simulink model "accelerr_test_drvr"  (Simulink 4.00)
settings: Solver=ode45  StartTime=0.0  StopTime=10.0  RelTol=1e-3
undefined symbols (not defined in the file or in its folder): DCM_B2L, DCM_L2E, skew
settings Model: Creator=mcar  LastModifiedBy=mcar  BlockReductionOpt=off

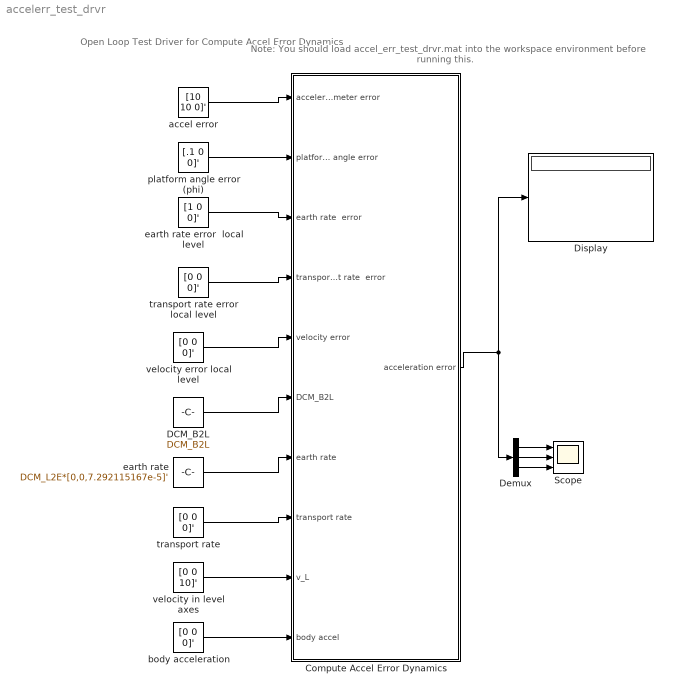
== system accelerr_test_drvr ==
  note: Open Loop Test Driver
      | for Compute Accel Error
      | Dynamics
  note: Note: You should load accel_err_test_drvr.mat into
      | the workspace environment before running this.
  Compute Accel Error Dynamics : Subsystem
      settings: RTWFcnNameOpts=Auto  RTWFileNameOpts=Auto
  DCM_B2L : Constant  Value=DCM_B2L  VectorParams1D=off
  Demux : Demux  Outputs=3  BusSelectionMode=off
  Display : Display
      settings: Format=short
  Scope : Scope  NumInputPorts=3
      settings: TimeRange=auto  YMin=-5~-5~-5  YMax=5~5~5  SaveToWorkspace=off  SaveName=ScopeData  LimitDataPoints=on  MaxDataPoints=5000
  accel error : Constant  Value=[10 10 0]'  VectorParams1D=off
  body acceleration : Constant  Value=[0 0 0]'  VectorParams1D=off
  earth rate : Constant  Value=DCM_L2E*[0,0,7.292115167e-5]'  VectorParams1D=off
  earth rate error  local level : Constant  Value=[1 0 0]'  VectorParams1D=off
  platform angle error (phi) : Constant  Value=[.1 0 0]'  VectorParams1D=off
  transport rate : Constant  Value=[0 0 0]'  VectorParams1D=off
  transport rate error local level : Constant  Value=[0 0 0]'  VectorParams1D=off
  velocity error local level : Constant  Value=[0 0 0]'  VectorParams1D=off
  velocity in level axes : Constant  Value=[0 0 10]'  VectorParams1D=off
  wires:
  body acceleration/1 -> Compute Accel Error Dynamics/10(body accel)
  velocity in level axes/1 -> Compute Accel Error Dynamics/9(v_L)
  transport rate/1 -> Compute Accel Error Dynamics/8(transport rate)
  earth rate/1 -> Compute Accel Error Dynamics/7(earth rate)
  DCM_B2L/1 -> Compute Accel Error Dynamics/6(DCM_B2L)
  velocity error local level/1 -> Compute Accel Error Dynamics/5(velocity error)
  transport rate error local level/1 -> Compute Accel Error Dynamics/4(transport rate  error)
  earth rate error  local level/1 -> Compute Accel Error Dynamics/3(earth rate  error)
  platform angle error (phi)/1 -> Compute Accel Error Dynamics/2(platform  angle error)
  accel error/1 -> Compute Accel Error Dynamics/1(accelerometer error)
  Compute Accel Error Dynamics/1(acceleration error) -> Demux/1, Display/1
  Demux/1 -> Scope/1
  Demux/2 -> Scope/2
  Demux/3 -> Scope/3

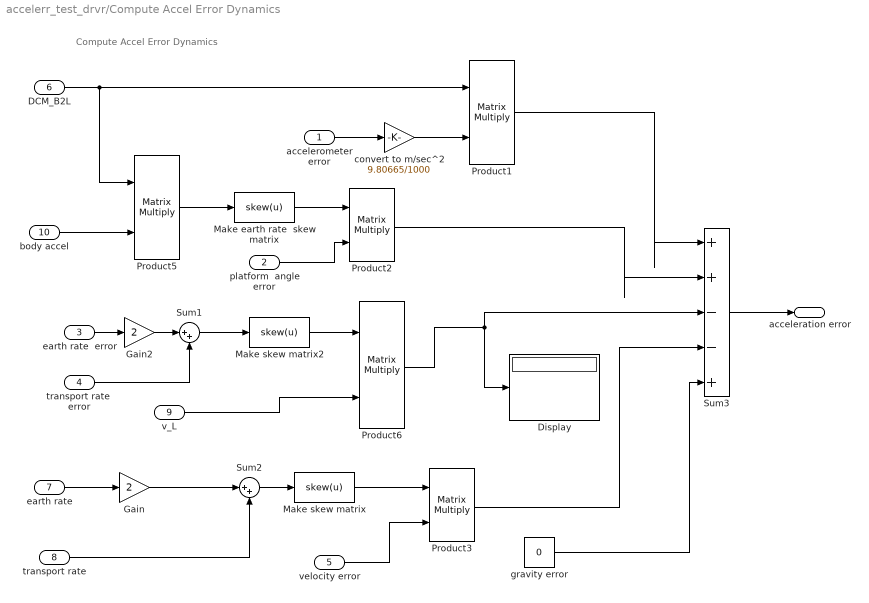
== system accelerr_test_drvr/Compute Accel Error Dynamics ==
  note: Compute Accel Error Dynamics
  accelerometer error : Inport  Port=1
  platform  angle error : Inport  Port=2
  earth rate  error : Inport  Port=3
  transport rate  error : Inport  Port=4
  velocity error : Inport  Port=5
  DCM_B2L : Inport  Port=6
  earth rate : Inport  Port=7
  transport rate : Inport  Port=8
  v_L : Inport  Port=9
  body accel : Inport  Port=10
  Display : Display
      settings: Format=short
  Gain : Gain  Gain=2  Multiplication=Element-wise(K.*u)  SaturateOnIntegerOverflow=on
  Gain2 : Gain  Gain=2  Multiplication=Element-wise(K.*u)  SaturateOnIntegerOverflow=on
  Make earth rate  skew matrix : MATLABFcn  MATLABFcn=skew(u)  OutputDimensions=-1  OutputSignalType=auto  Output1D=off
  Make skew matrix : MATLABFcn  MATLABFcn=skew(u)  OutputDimensions=-1  OutputSignalType=auto  Output1D=off
  Make skew matrix2 : MATLABFcn  MATLABFcn=skew(u)  OutputDimensions=-1  OutputSignalType=auto  Output1D=off
  Product{1..3,5..6} (5 alike) : Product  Inputs=2  Multiplication=Matrix(*)  SaturateOnIntegerOverflow=on
  Sum1 : Sum  Inputs=|++  SaturateOnIntegerOverflow=on
  Sum2 : Sum  Inputs=|++  SaturateOnIntegerOverflow=on
  Sum3 : Sum  Inputs=|++--+  SaturateOnIntegerOverflow=on
  convert to m/sec^2 : Gain  Gain=9.80665/1000  Multiplication=Element-wise(K.*u)  SaturateOnIntegerOverflow=on
  gravity error : Constant  Value=0
  acceleration error : Outport  Port=1
  wires:
  accelerometer error/1 -> convert to m/sec^2/1
  Make earth rate  skew matrix/1 -> Product2/1
  platform  angle error/1 -> Product2/2
  Gain/1 -> Sum2/1
  Sum2/1 -> Make skew matrix/1
  Make skew matrix/1 -> Product3/1
  velocity error/1 -> Product3/2
  earth rate  error/1 -> Gain2/1
  Gain2/1 -> Sum1/1
  transport rate  error/1 -> Sum1/2
  Sum1/1 -> Make skew matrix2/1
  Sum3/1 -> acceleration error/1
  Product1/1 -> Sum3/1
  Product2/1 -> Sum3/2
  gravity error/1 -> Sum3/5
  Product3/1 -> Sum3/4
  Product6/1 -> Sum3/3, Display/1
  DCM_B2L/1 -> Product1/1, Product5/1
  earth rate/1 -> Gain/1
  transport rate/1 -> Sum2/2
  v_L/1 -> Product6/2
  convert to m/sec^2/1 -> Product1/2
  body accel/1 -> Product5/2
  Product5/1 -> Make earth rate  skew matrix/1
  Make skew matrix2/1 -> Product6/1
